simulink library "Camera_Frame_Definitions"  (R2025a)
settings: Solver=VariableStepAuto  StartTime=0.0  StopTime=10.0  RelTol=1e-3
values from neighbouring files (symbols this model uses):
  Camera = sm_car_define_camera(camera_param)    [sm_car_define_camera_sedan.m]
undefined symbols (not defined in the file or in its folder): X, Y, Z
libraries: sm_lib x40, $bdroot x30, nesl_utility x3
Description:
  | Component of Simscape Vehicle Templates Library
  | 
  | Copyright 2018-2026 The MathWorks, Inc.
settings Model: Creator=smiller  LastModifiedBy=smiller
settings SolverCC: AlgebraicLoopSolver=TrustRegion
settings DataIOCC: ReturnWorkspaceOutputs=off
settings OptimizationCC: LifeSpan=inf
settings DebuggingCC: UnconnectedInputMsg=warning  UnconnectedOutputMsg=warning  UnconnectedLineMsg=warning  SFExecutionAtInitializationDiag=none  ArithmeticOperatorsInVariantConditions=warning
settings ModelReferenceCC: EnableRefExpFcnMdlSchedulingChecks=on
settings SFSimCC: CustomCodeUndefinedFunction=UseInterfaceOnly
settings RTWCC: GPUComputeCapability=3.5
settings CodeAppCC: StateflowObjectComments=on

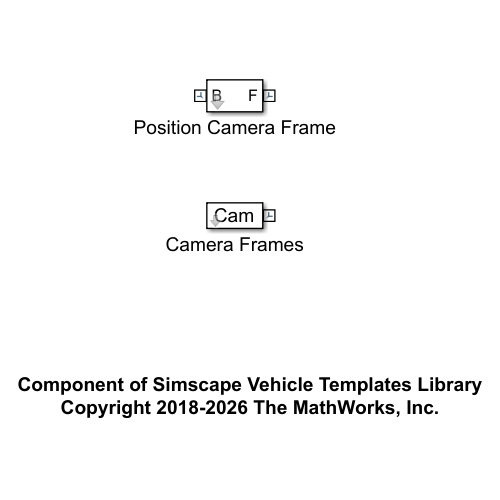
[thumbnail: Simulink's stored preview of the top-level diagram]
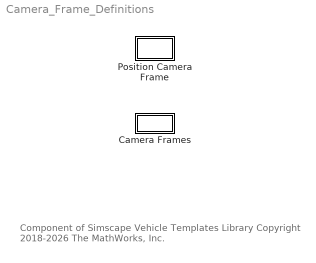
== system Camera_Frame_Definitions ==
  note: Component of Simscape Vehicle Templates Library
      | Copyright 2018-2026 The MathWorks, Inc.
  Camera Frames : Subsystem  mask(Camera Frame Definitions){Camera=Camera, popup_dolly_camera=Off}
      mask prompts: popup_dolly_camera "Dolly Camera"
      mask help: Defines set of camera frames surrounding vehicle. Frames are used to define visualization viewpoints for animation of simulation results.
      mask init:
      | if(verLessThan('matlab','9.5'))
      |   set_param([gcb '/Dolly Camera'],'OverrideUsingVariant',get_param(gcb,'popup_dolly_camera'));
      | else
      |   set_param([gcb '/Dolly Camera'],'LabelModeActiveChoice',get_param(gcb,'popup_dolly_camera'));
      | end
      mask TypeOptions popup_dolly_camera: Off | XYZ
      mask Display: disp('Cam')
  Position Camera Frame : Subsystem  mask(Define Camera Frame){CF=Camera.Rear}
      mask prompts: CF "Camera Frame Data (structure)"
      mask help: Sets frame position and orientation for camera frame. Data structure provides cartesian location and orientation. Orientation is intrinsic rotation of yaw-pitch-roll.

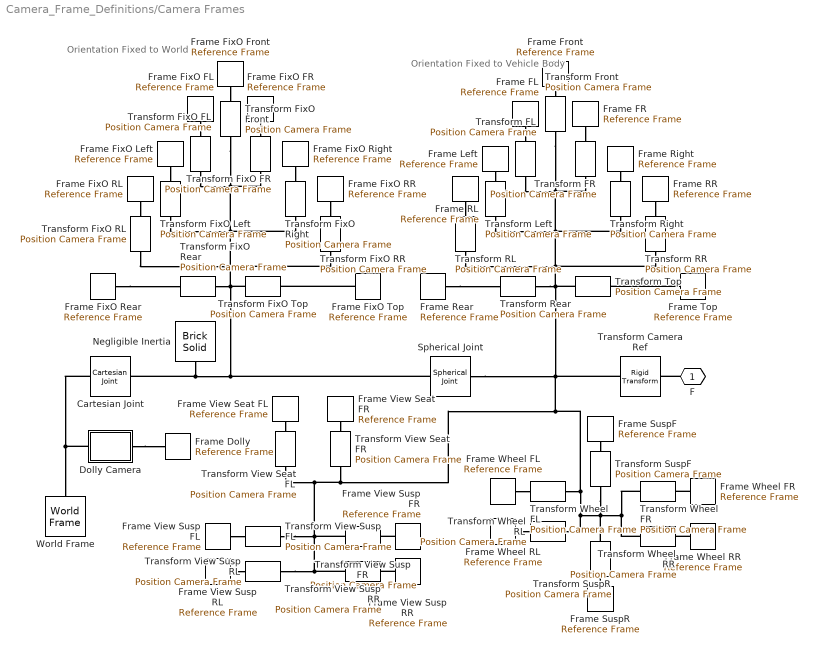
== system Camera_Frame_Definitions/Camera Frames ==
  note: Orientation Fixed to Vehicle Body
  note: Orientation Fixed to World
  Cartesian Joint : sm_lib/Joints/Cartesian Joint  JointMode=Normal  CompositeWrenchDir=FollowerOnBase  CompositeWrenchFrame=BaseFrame  SenseConstraintForce=off  SenseConstraintTorque=off  SenseTotalForce=off  SenseTotalTorque=off  PxPositionTargetSpecify=off  PxPositionTargetPriority=High  PxPositionTargetValue=0  PxPositionTargetValueUnits=m  PxVelocityTargetSpecify=off  PxVelocityTargetPriority=High  PxVelocityTargetValue=0  PxVelocityTargetValueUnits=m/s  PxEquilibriumPosition=0  PxEquilibriumPositionUnits=m  PxSpringStiffness=0  PxSpringStiffnessUnits=N/m  PxDampingCoefficient=0  PxDampingCoefficientUnits=N/(m/s)  PxLowerLimitSpecify=off  PxLowerLimitBound=-1  PxLowerLimitBoundUnits=m  PxLowerLimitStiffness=1e6  PxLowerLimitStiffnessUnits=N/m  PxLowerLimitDamping=1e3  PxLowerLimitDampingUnits=N/(m/s)  PxLowerLimitTransitionRegionWidth=1e-4  PxLowerLimitTransitionRegionWidthUnits=m  PxUpperLimitSpecify=off  PxUpperLimitBound=1  PxUpperLimitBoundUnits=m  PxUpperLimitStiffness=1e6  PxUpperLimitStiffnessUnits=N/m  PxUpperLimitDamping=1e3  PxUpperLimitDampingUnits=N/(m/s)  PxUpperLimitTransitionRegionWidth=1e-4  PxUpperLimitTransitionRegionWidthUnits=m  PxTorqueActuationMode=NoTorque  PxMotionActuationMode=ComputedMotion  PxSensePosition=off  PxSenseVelocity=off  PxSenseAcceleration=off  PxSenseTorqueForce=off  PxSenseLowerLimitTorqueForce=off  PxSenseUpperLimitTorqueForce=off  PyPositionTargetSpecify=off  PyPositionTargetPriority=High  PyPositionTargetValue=0  PyPositionTargetValueUnits=m  PyVelocityTargetSpecify=off  PyVelocityTargetPriority=High  PyVelocityTargetValue=0  PyVelocityTargetValueUnits=m/s  PyEquilibriumPosition=0  PyEquilibriumPositionUnits=m  PySpringStiffness=0  PySpringStiffnessUnits=N/m  PyDampingCoefficient=0  PyDampingCoefficientUnits=N/(m/s)  PyLowerLimitSpecify=off  PyLowerLimitBound=-1  PyLowerLimitBoundUnits=m  PyLowerLimitStiffness=1e6  PyLowerLimitStiffnessUnits=N/m  PyLowerLimitDamping=1e3  PyLowerLimitDampingUnits=N/(m/s)  PyLowerLimitTransitionRegionWidth=1e-4  PyLowerLimitTransitionRegionWidthUnits=m  PyUpperLimitSpecify=off  PyUpperLimitBound=1  PyUpperLimitBoundUnits=m  PyUpperLimitStiffness=1e6  PyUpperLimitStiffnessUnits=N/m  PyUpperLimitDamping=1e3  PyUpperLimitDampingUnits=N/(m/s)  PyUpperLimitTransitionRegionWidth=1e-4  PyUpperLimitTransitionRegionWidthUnits=m  PyTorqueActuationMode=NoTorque  PyMotionActuationMode=ComputedMotion  PySensePosition=off  PySenseVelocity=off  PySenseAcceleration=off  PySenseTorqueForce=off  PySenseLowerLimitTorqueForce=off  PySenseUpperLimitTorqueForce=off  PzPositionTargetSpecify=off  PzPositionTargetPriority=High  PzPositionTargetValue=0  PzPositionTargetValueUnits=m  PzVelocityTargetSpecify=off  PzVelocityTargetPriority=High  PzVelocityTargetValue=0  PzVelocityTargetValueUnits=m/s  PzEquilibriumPosition=0  PzEquilibriumPositionUnits=m  PzSpringStiffness=0  PzSpringStiffnessUnits=N/m  PzDampingCoefficient=0  PzDampingCoefficientUnits=N/(m/s)  PzLowerLimitSpecify=off  PzLowerLimitBound=-1  PzLowerLimitBoundUnits=m  PzLowerLimitStiffness=1e6  PzLowerLimitStiffnessUnits=N/m  PzLowerLimitDamping=1e3  PzLowerLimitDampingUnits=N/(m/s)  PzLowerLimitTransitionRegionWidth=1e-4  PzLowerLimitTransitionRegionWidthUnits=m  PzUpperLimitSpecify=off  PzUpperLimitBound=1  PzUpperLimitBoundUnits=m  PzUpperLimitStiffness=1e6  PzUpperLimitStiffnessUnits=N/m  PzUpperLimitDamping=1e3  PzUpperLimitDampingUnits=N/(m/s)  PzUpperLimitTransitionRegionWidth=1e-4  PzUpperLimitTransitionRegionWidthUnits=m  PzTorqueActuationMode=NoTorque  PzMotionActuationMode=ComputedMotion  PzSensePosition=off  PzSenseVelocity=off  PzSenseAcceleration=off  PzSenseTorqueForce=off  PzSenseLowerLimitTorqueForce=off  PzSenseUpperLimitTorqueForce=off
  Dolly Camera : Subsystem  Variant=on  VariantControlMode=label  VariantControl=Variant1  LabelModeActiveChoice=Off
      settings: AttributesFormatString=%<ActiveVariant>
      mask Display: disp(' ');
  Frame Dolly : sm_lib/Frames and Transforms/Reference Frame
  Frame FL : sm_lib/Frames and Transforms/Reference Frame
  Frame FR : sm_lib/Frames and Transforms/Reference Frame
  Frame FixO FL : sm_lib/Frames and Transforms/Reference Frame
  Frame FixO FR : sm_lib/Frames and Transforms/Reference Frame
  Frame FixO Front : sm_lib/Frames and Transforms/Reference Frame
  Frame FixO Left : sm_lib/Frames and Transforms/Reference Frame
  Frame FixO RL : sm_lib/Frames and Transforms/Reference Frame
  Frame FixO RR : sm_lib/Frames and Transforms/Reference Frame
  Frame FixO Rear : sm_lib/Frames and Transforms/Reference Frame
  Frame FixO Right : sm_lib/Frames and Transforms/Reference Frame
  Frame FixO Top : sm_lib/Frames and Transforms/Reference Frame
  Frame Front : sm_lib/Frames and Transforms/Reference Frame
  Frame Left : sm_lib/Frames and Transforms/Reference Frame
  Frame RL : sm_lib/Frames and Transforms/Reference Frame
  Frame RR : sm_lib/Frames and Transforms/Reference Frame
  Frame Rear : sm_lib/Frames and Transforms/Reference Frame
  Frame Right : sm_lib/Frames and Transforms/Reference Frame
  Frame SuspF : sm_lib/Frames and Transforms/Reference Frame
  Frame SuspR : sm_lib/Frames and Transforms/Reference Frame
  Frame Top : sm_lib/Frames and Transforms/Reference Frame
  Frame View Seat FL : sm_lib/Frames and Transforms/Reference Frame
  Frame View Seat FR : sm_lib/Frames and Transforms/Reference Frame
  Frame View Susp FL : sm_lib/Frames and Transforms/Reference Frame
  Frame View Susp FR : sm_lib/Frames and Transforms/Reference Frame
  Frame View Susp RL : sm_lib/Frames and Transforms/Reference Frame
  Frame View Susp RR : sm_lib/Frames and Transforms/Reference Frame
  Frame Wheel FL : sm_lib/Frames and Transforms/Reference Frame
  Frame Wheel FR : sm_lib/Frames and Transforms/Reference Frame
  Frame Wheel RL : sm_lib/Frames and Transforms/Reference Frame
  Frame Wheel RR : sm_lib/Frames and Transforms/Reference Frame
  Negligible Inertia : sm_lib/Body Elements/Brick Solid  BrickDimensions=[1 1 1]*1e-3  BrickDimensionsUnits=m  ExportEntireGeometry=off  InertiaType=PointMass  BasedOnType=Density  Density=1000  DensityUnits=kg/m^3  Mass=1e-6  MassUnits=kg  CenterOfMass=[0 0 0]  CenterOfMassUnits=m  MomentsOfInertia=[1 1 1]  MomentsOfInertiaUnits=kg*m^2  ProductsOfInertia=[1 1 1]  ProductsOfInertiaUnits=kg*m^2  GraphicType=FromGeometry  MarkerShape=Sphere  MarkerSize=10  GraphicVisPropType=SimpleVisualProperties  GraphicDiffuseColor=[0.5 0.5 0.5]  GraphicOpacity=1.0  GraphicSpecularColor=[0.5 0.5 0.5 1.0]  GraphicAmbientColor=[0.15 0.15 0.15 1.0]  GraphicEmissiveColor=[0.0 0.0 0.0 1.0]  GraphicShininess=75  DoExposeReferenceFrame=on  SerializedFrames=<Frames/>
  Spherical Joint : sm_lib/Joints/Spherical Joint  JointMode=Normal  CompositeWrenchDir=FollowerOnBase  CompositeWrenchFrame=BaseFrame  SenseConstraintForce=off  SenseConstraintTorque=off  SenseTotalForce=off  SenseTotalTorque=off  PositionTargetSpecify=off  PositionTargetPriority=High  PositionTargetRotationMethod=None  PositionTargetFollAlignAxisA=+X  PositionTargetBaseAlignAxisA=+Y  PositionTargetFollAlignAxisB=+Y  PositionTargetBaseAlignAxisB=+Z  PositionTargetRotationStandardAxis=+Z  PositionTargetRotationAngle=0.0  PositionTargetRotationAngleUnits=deg  PositionTargetRotationArbitraryAxis=[0 0 1]  PositionTargetRotationSequenceAxes=FollowerAxes  PositionTargetRotationSequence=XYX  PositionTargetRotationSequenceAngles=[0 0 0]  PositionTargetRotationSequenceAnglesUnits=deg  PositionTargetRotationMatrix=[1 0 0; 0 1 0; 0 0 1]  PositionTargetQuaternion=[1 0 0 0]  VelocityTargetSpecify=off  VelocityTargetPriority=High  VelocityTargetValue=[0 0 0]  VelocityTargetValueUnits=deg/s  VelocityTargetInFollowerFrame=on  EqPosRotationMethod=None  EqPosFollAlignAxisA=+X  EqPosBaseAlignAxisA=+Y  EqPosFollAlignAxisB=+Y  EqPosBaseAlignAxisB=+Z  EqPosRotationStandardAxis=+Z  EqPosRotationAngle=0.0  EqPosRotationAngleUnits=deg  EqPosRotationArbitraryAxis=[0 0 1]  EqPosRotationSequenceAxes=FollowerAxes  EqPosRotationSequence=XYX  EqPosRotationSequenceAngles=[0 0 0]  EqPosRotationSequenceAnglesUnits=deg  EqPosRotationMatrix=[1 0 0; 0 1 0; 0 0 1]  EqPosQuaternion=[1 0 0 0]  SpringStiffness=0  SpringStiffnessUnits=N*m/deg  DampingCoefficient=0  DampingCoefficientUnits=N*m/(deg/s)  LowerLimitSpecify=off  LowerLimitBound=15  LowerLimitBoundUnits=deg  LowerLimitStiffness=1e4  LowerLimitStiffnessUnits=N*m/deg  LowerLimitDamping=10  LowerLimitDampingUnits=N*m/(deg/s)  LowerLimitTransitionRegionWidth=0.1  LowerLimitTransitionRegionWidthUnits=deg  UpperLimitSpecify=off  UpperLimitBound=45  UpperLimitBoundUnits=deg  UpperLimitStiffness=1e4  UpperLimitStiffnessUnits=N*m/deg  UpperLimitDamping=10  UpperLimitDampingUnits=N*m/(deg/s)  UpperLimitTransitionRegionWidth=0.1  UpperLimitTransitionRegionWidthUnits=deg  TorqueActuationMode=NoTorque  ActuateTorqueX=off  ActuateTorqueY=off  ActuateTorqueZ=off  ActuateTorque=off  ActuationFrame=BaseFrame  SensePosition=off  SenseVelocityX=off  SenseVelocityY=off  SenseVelocityZ=off  SenseVelocity=off  SenseAccelerationX=off  SenseAccelerationY=off  SenseAccelerationZ=off  SenseAcceleration=off  SenseLowerLimitTorqueMag=off  SenseUpperLimitTorqueMag=off  SensingFrame=BaseFrame
  Transform Camera Ref : sm_lib/Frames and Transforms/Rigid Transform  RotationMethod=RotationSequence  FollAlignAxisA=+X  BaseAlignAxisA=+Y  FollAlignAxisB=+Y  BaseAlignAxisB=+Z  RotationStandardAxis=+Z  RotationAngle=0.0  RotationAngleUnits=deg  RotationArbitraryAxis=[0 0 1]  RotationSequenceAxes=FollowerAxes  RotationSequence=ZYX  RotationSequenceAngles=[Camera.Offset.a.Value(3) Camera.Offset.a.Value(2) Camera.Offset.a.Value(1)]  RotationSequenceAnglesUnits=deg  RotationMatrix=[1 0 0; 0 1 0; 0 0 1]  Quaternion=[1 0 0 0]  TranslationMethod=Cartesian  TranslationCartesianOffset=Camera.Offset.s.Value  TranslationCartesianOffsetUnits=m  TranslationStandardAxis=+Z  TranslationStandardOffset=0  TranslationStandardOffsetUnits=m  TranslationROffset=0  TranslationROffsetUnits=m  TranslationThetaOffset=0  TranslationThetaOffsetUnits=deg  TranslationZOffset=0  TranslationZOffsetUnits=m
  Transform FL : $bdroot/Position Camera Frame  CF=Camera.FL
  Transform FR : $bdroot/Position Camera Frame  CF=Camera.FR
  Transform FixO FL : $bdroot/Position Camera Frame  CF=Camera.FL
  Transform FixO FR : $bdroot/Position Camera Frame  CF=Camera.FR
  Transform FixO Front : $bdroot/Position Camera Frame  CF=Camera.Front
  Transform FixO Left : $bdroot/Position Camera Frame  CF=Camera.Left
  Transform FixO RL : $bdroot/Position Camera Frame  CF=Camera.RL
  Transform FixO RR : $bdroot/Position Camera Frame  CF=Camera.RR
  Transform FixO Rear : $bdroot/Position Camera Frame  CF=Camera.Rear
  Transform FixO Right : $bdroot/Position Camera Frame  CF=Camera.Right
  Transform FixO Top : $bdroot/Position Camera Frame  CF=Camera.Top
  Transform Front : $bdroot/Position Camera Frame  CF=Camera.Front
  Transform Left : $bdroot/Position Camera Frame  CF=Camera.Left
  Transform RL : $bdroot/Position Camera Frame  CF=Camera.RL
  Transform RR : $bdroot/Position Camera Frame  CF=Camera.RR
  Transform Rear : $bdroot/Position Camera Frame  CF=Camera.Rear
  Transform Right : $bdroot/Position Camera Frame  CF=Camera.Right
  Transform SuspF : $bdroot/Position Camera Frame  CF=Camera.SuspF
  Transform SuspR : $bdroot/Position Camera Frame  CF=Camera.SuspR
  Transform Top : $bdroot/Position Camera Frame  CF=Camera.Top
  Transform View Seat FL : $bdroot/Position Camera Frame  CF=Camera.View_SeatFL
  Transform View Seat FR : $bdroot/Position Camera Frame  CF=Camera.View_SeatFR
  Transform View Susp FL : $bdroot/Position Camera Frame  CF=Camera.View_SuspFL
  Transform View Susp FR : $bdroot/Position Camera Frame  CF=Camera.View_SuspFR
  Transform View Susp RL : $bdroot/Position Camera Frame  CF=Camera.View_SuspRL
  Transform View Susp RR : $bdroot/Position Camera Frame  CF=Camera.View_SuspRR
  Transform Wheel FL : $bdroot/Position Camera Frame  CF=Camera.Wheel_FL
  Transform Wheel FR : $bdroot/Position Camera Frame  CF=Camera.Wheel_FR
  Transform Wheel RL : $bdroot/Position Camera Frame  CF=Camera.Wheel_RL
  Transform Wheel RR : $bdroot/Position Camera Frame  CF=Camera.Wheel_RR
  World Frame : sm_lib/Frames and Transforms/World Frame
  F : PMIOPort  Side=Right
  connections:
  F/RConn1 -- Transform Camera Ref/LConn1
  Transform View Susp FR/LConn1 -- Transform View Susp RL/LConn1 -- Transform View Susp RR/LConn1 -- Transform View Seat FR/LConn1 -- Transform Wheel RR/LConn1 -- Transform Wheel FR/LConn1 -- Transform SuspR/LConn1 -- Transform SuspF/LConn1 -- Transform Wheel RL/LConn1 -- Transform Wheel FL/LConn1 -- Spherical Joint/RConn1 -- Transform Camera Ref/RConn1 -- Transform Top/LConn1 -- Transform RL/LConn1 -- Transform RR/LConn1 -- Transform Left/LConn1 -- Transform Right/LConn1 -- Transform FR/LConn1 -- Transform Front/LConn1 -- Transform FL/LConn1 -- Transform Rear/LConn1 -- Transform View Seat FL/LConn1 -- Transform View Susp FL/LConn1
  Dolly Camera/LConn1 -- Cartesian Joint/LConn1 -- World Frame/RConn1
  Negligible Inertia/RConn1 -- Cartesian Joint/RConn1 -- Spherical Joint/LConn1 -- Transform FixO Rear/LConn1 -- Transform FixO Top/LConn1 -- Transform FixO FL/LConn1 -- Transform FixO Front/LConn1 -- Transform FixO FR/LConn1 -- Transform FixO Right/LConn1 -- Transform FixO Left/LConn1 -- Transform FixO RR/LConn1 -- Transform FixO RL/LConn1
  Frame FixO FR/RConn1 -- Transform FixO FR/RConn1
  Frame FixO Right/RConn1 -- Transform FixO Right/RConn1
  Frame FixO RR/RConn1 -- Transform FixO RR/RConn1
  Frame FixO RL/RConn1 -- Transform FixO RL/RConn1
  Frame FixO Left/RConn1 -- Transform FixO Left/RConn1
  Frame FixO FL/RConn1 -- Transform FixO FL/RConn1
  Frame FixO Top/RConn1 -- Transform FixO Top/RConn1
  Frame FixO Front/RConn1 -- Transform FixO Front/RConn1
  Frame FixO Rear/RConn1 -- Transform FixO Rear/RConn1
  Frame Rear/RConn1 -- Transform Rear/RConn1
  Frame Top/RConn1 -- Transform Top/RConn1
  Frame Left/RConn1 -- Transform Left/RConn1
  Frame FL/RConn1 -- Transform FL/RConn1
  Frame RL/RConn1 -- Transform RL/RConn1
  Frame Right/RConn1 -- Transform Right/RConn1
  Frame FR/RConn1 -- Transform FR/RConn1
  Frame RR/RConn1 -- Transform RR/RConn1
  Frame Front/RConn1 -- Transform Front/RConn1
  Frame SuspF/RConn1 -- Transform SuspF/RConn1
  Frame SuspR/RConn1 -- Transform SuspR/RConn1
  Frame Wheel FR/RConn1 -- Transform Wheel FR/RConn1
  Frame Wheel RR/RConn1 -- Transform Wheel RR/RConn1
  Frame Wheel FL/RConn1 -- Transform Wheel FL/RConn1
  Frame Wheel RL/RConn1 -- Transform Wheel RL/RConn1
  Frame View Seat FL/RConn1 -- Transform View Seat FL/RConn1
  Frame View Seat FR/RConn1 -- Transform View Seat FR/RConn1
  Frame View Susp FL/RConn1 -- Transform View Susp FL/RConn1
  Frame View Susp FR/RConn1 -- Transform View Susp FR/RConn1
  Frame View Susp RR/RConn1 -- Transform View Susp RR/RConn1
  Frame View Susp RL/RConn1 -- Transform View Susp RL/RConn1
  Dolly Camera/RConn1 -- Frame Dolly/RConn1

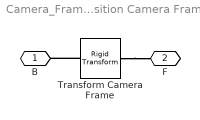
== system Camera_Frame_Definitions/Position Camera Frame ==
  Transform Camera Frame : sm_lib/Frames and Transforms/Rigid Transform  RotationMethod=RotationSequence  FollAlignAxisA=+X  BaseAlignAxisA=+Y  FollAlignAxisB=+Y  BaseAlignAxisB=+Z  RotationStandardAxis=+Z  RotationAngle=0.0  RotationAngleUnits=deg  RotationArbitraryAxis=[0 0 1]  RotationSequenceAxes=FollowerAxes  RotationSequence=ZYX  RotationSequenceAngles=CF.a.Value(3:-1:1)  RotationSequenceAnglesUnits=deg  RotationMatrix=[1 0 0; 0 1 0; 0 0 1]  Quaternion=[1 0 0 0]  TranslationMethod=Cartesian  TranslationCartesianOffset=CF.s.Value  TranslationCartesianOffsetUnits=m  TranslationStandardAxis=+Z  TranslationStandardOffset=0  TranslationStandardOffsetUnits=m  TranslationROffset=0  TranslationROffsetUnits=m  TranslationThetaOffset=0  TranslationThetaOffsetUnits=deg  TranslationZOffset=0  TranslationZOffsetUnits=m
  B : PMIOPort  Side=Left
  F : PMIOPort  Port=2  Side=Right
  connections:
  Transform Camera Frame/LConn1 -- B/RConn1
  Transform Camera Frame/RConn1 -- F/RConn1

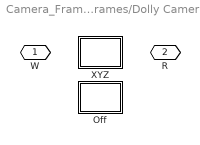
== system Camera_Frame_Definitions/Camera Frames/Dolly Camera ==
  Off : Subsystem  VariantControl=Off  mask{tvec=Camera.Dolly_Cam.tvec.Value, xvec=Camera.Dolly_Cam.xvec.Value, yvec=Camera.Dolly_Cam.yvec.Value, zvec=Camera.Dolly_Cam.zvec.Value, s=Camera.Dolly_Cam.s.Value, a=Camera.Dolly_Cam.a.Value}
      mask prompts: tvec "Time Vector (s)"; xvec "X Vector (m)"; yvec "Y Vector (m)"; zvec "Z Vector (m)"; s "Camera Offset [xyz] (m)"; a "Camera Orientation [Roll-Pitch-Yaw] (deg)"
  XYZ : Subsystem  VariantControl=XYZ  mask{tvec=Camera.Dolly_Cam.tvec.Value, xvec=Camera.Dolly_Cam.xvec.Value, yvec=Camera.Dolly_Cam.yvec.Value, zvec=Camera.Dolly_Cam.zvec.Value, s=Camera.Dolly_Cam.s.Value, a=Camera.Dolly_Cam.a.Value}
      mask prompts: tvec "Time Vector (s)"; xvec "X Vector (m)"; yvec "Y Vector (m)"; zvec "Z Vector (m)"; s "Camera Offset [xyz] (m)"; a "Camera Orientation [Roll-Pitch-Yaw] (deg)"
  " W" : PMIOPort  Side=Left
  " R" : PMIOPort  Port=2  Side=Right

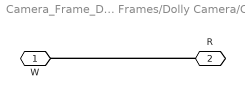
== system Camera_Frame_Definitions/Camera Frames/Dolly Camera/Off ==
  W : PMIOPort  Side=Left
  R : PMIOPort  Port=2  Side=Right
  connections:
  R/RConn1 -- W/RConn1

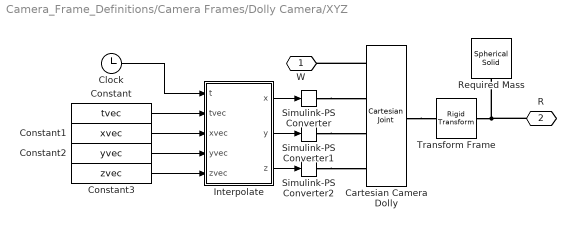
== system Camera_Frame_Definitions/Camera Frames/Dolly Camera/XYZ ==
  Cartesian Camera Dolly : sm_lib/Joints/Cartesian Joint  JointMode=Normal  CompositeWrenchDir=FollowerOnBase  CompositeWrenchFrame=BaseFrame  SenseConstraintForce=off  SenseConstraintTorque=off  SenseTotalForce=off  SenseTotalTorque=off  PxPositionTargetSpecify=on  PxPositionTargetPriority=High  PxPositionTargetValue=xvec(1)  PxPositionTargetValueUnits=m  PxVelocityTargetSpecify=off  PxVelocityTargetPriority=High  PxVelocityTargetValue=0  PxVelocityTargetValueUnits=m/s  PxEquilibriumPosition=0  PxEquilibriumPositionUnits=m  PxSpringStiffness=0  PxSpringStiffnessUnits=N/m  PxDampingCoefficient=0  PxDampingCoefficientUnits=N/(m/s)  PxLowerLimitSpecify=off  PxLowerLimitBound=-1  PxLowerLimitBoundUnits=m  PxLowerLimitStiffness=1e6  PxLowerLimitStiffnessUnits=N/m  PxLowerLimitDamping=1e3  PxLowerLimitDampingUnits=N/(m/s)  PxLowerLimitTransitionRegionWidth=1e-4  PxLowerLimitTransitionRegionWidthUnits=m  PxUpperLimitSpecify=off  PxUpperLimitBound=1  PxUpperLimitBoundUnits=m  PxUpperLimitStiffness=1e6  PxUpperLimitStiffnessUnits=N/m  PxUpperLimitDamping=1e3  PxUpperLimitDampingUnits=N/(m/s)  PxUpperLimitTransitionRegionWidth=1e-4  PxUpperLimitTransitionRegionWidthUnits=m  PxTorqueActuationMode=ComputedTorque  PxMotionActuationMode=InputMotion  PxSensePosition=off  PxSenseVelocity=off  PxSenseAcceleration=off  PxSenseTorqueForce=off  PxSenseLowerLimitTorqueForce=off  PxSenseUpperLimitTorqueForce=off  PyPositionTargetSpecify=on  PyPositionTargetPriority=High  PyPositionTargetValue=yvec(1)  PyPositionTargetValueUnits=m  PyVelocityTargetSpecify=off  PyVelocityTargetPriority=High  PyVelocityTargetValue=0  PyVelocityTargetValueUnits=m/s  PyEquilibriumPosition=0  PyEquilibriumPositionUnits=m  PySpringStiffness=0  PySpringStiffnessUnits=N/m  PyDampingCoefficient=0  PyDampingCoefficientUnits=N/(m/s)  PyLowerLimitSpecify=off  PyLowerLimitBound=-1  PyLowerLimitBoundUnits=m  PyLowerLimitStiffness=1e6  PyLowerLimitStiffnessUnits=N/m  PyLowerLimitDamping=1e3  PyLowerLimitDampingUnits=N/(m/s)  PyLowerLimitTransitionRegionWidth=1e-4  PyLowerLimitTransitionRegionWidthUnits=m  PyUpperLimitSpecify=off  PyUpperLimitBound=1  PyUpperLimitBoundUnits=m  PyUpperLimitStiffness=1e6  PyUpperLimitStiffnessUnits=N/m  PyUpperLimitDamping=1e3  PyUpperLimitDampingUnits=N/(m/s)  PyUpperLimitTransitionRegionWidth=1e-4  PyUpperLimitTransitionRegionWidthUnits=m  PyTorqueActuationMode=ComputedTorque  PyMotionActuationMode=InputMotion  PySensePosition=off  PySenseVelocity=off  PySenseAcceleration=off  PySenseTorqueForce=off  PySenseLowerLimitTorqueForce=off  PySenseUpperLimitTorqueForce=off  PzPositionTargetSpecify=on  PzPositionTargetPriority=High  PzPositionTargetValue=zvec(1)  PzPositionTargetValueUnits=m  PzVelocityTargetSpecify=off  PzVelocityTargetPriority=High  PzVelocityTargetValue=0  PzVelocityTargetValueUnits=m/s  PzEquilibriumPosition=0  PzEquilibriumPositionUnits=m  PzSpringStiffness=0  PzSpringStiffnessUnits=N/m  PzDampingCoefficient=0  PzDampingCoefficientUnits=N/(m/s)  PzLowerLimitSpecify=off  PzLowerLimitBound=-1  PzLowerLimitBoundUnits=m  PzLowerLimitStiffness=1e6  PzLowerLimitStiffnessUnits=N/m  PzLowerLimitDamping=1e3  PzLowerLimitDampingUnits=N/(m/s)  PzLowerLimitTransitionRegionWidth=1e-4  PzLowerLimitTransitionRegionWidthUnits=m  PzUpperLimitSpecify=off  PzUpperLimitBound=1  PzUpperLimitBoundUnits=m  PzUpperLimitStiffness=1e6  PzUpperLimitStiffnessUnits=N/m  PzUpperLimitDamping=1e3  PzUpperLimitDampingUnits=N/(m/s)  PzUpperLimitTransitionRegionWidth=1e-4  PzUpperLimitTransitionRegionWidthUnits=m  PzTorqueActuationMode=ComputedTorque  PzMotionActuationMode=InputMotion  PzSensePosition=off  PzSenseVelocity=off  PzSenseAcceleration=off  PzSenseTorqueForce=off  PzSenseLowerLimitTorqueForce=off  PzSenseUpperLimitTorqueForce=off
  Clock : Clock
  Constant : Constant  Value=tvec
  Constant1 : Constant  Value=xvec
  Constant2 : Constant  Value=yvec
  Constant3 : Constant  Value=zvec
  Interpolate : MATLAB Function  TreatAsAtomicUnit=on
  Required Mass : sm_lib/Body Elements/Spherical Solid  SphereRadius=0.05  SphereRadiusUnits=m  ExportEntireGeometry=off  InertiaType=CalculateFromGeometry  BasedOnType=Density  Density=1000  DensityUnits=kg/m^3  Mass=1  MassUnits=kg  CenterOfMass=[0 0 0]  CenterOfMassUnits=m  MomentsOfInertia=[1 1 1]  MomentsOfInertiaUnits=kg*m^2  ProductsOfInertia=[0 0 0]  ProductsOfInertiaUnits=kg*m^2  GraphicType=FromGeometry  MarkerShape=Sphere  MarkerSize=10  GraphicVisPropType=SimpleVisualProperties  GraphicDiffuseColor=[0.2 1.0 0.0]  GraphicOpacity=0  GraphicSpecularColor=[0.5 0.5 0.5 1.0]  GraphicAmbientColor=[0.15 0.15 0.15 1.0]  GraphicEmissiveColor=[0.0 0.0 0.0 1.0]  GraphicShininess=75  DoExposeReferenceFrame=on  SerializedFrames=<Frames/>
  Simulink-PS Converter : nesl_utility/Simulink-PS Converter  PhysicalDomain=network_engine_domain  SubClassName=ps_input  LeftPortType=input  RightPortType=output  PseudoPeriodic=off  Frequencies=[]  NoiseDistribution=none  NoiseParameters=[]  Unit=1  AffineConversion=off  FilteringAndDerivatives=filter  SimscapeFilterOrder=2  InputFilterTimeConstant=0.1  UdotUserProvided=1
  Simulink-PS Converter1 : nesl_utility/Simulink-PS Converter  PhysicalDomain=network_engine_domain  SubClassName=ps_input  LeftPortType=input  RightPortType=output  PseudoPeriodic=off  Frequencies=[]  NoiseDistribution=none  NoiseParameters=[]  Unit=1  AffineConversion=off  FilteringAndDerivatives=filter  SimscapeFilterOrder=2  InputFilterTimeConstant=0.1  UdotUserProvided=1
  Simulink-PS Converter2 : nesl_utility/Simulink-PS Converter  PhysicalDomain=network_engine_domain  SubClassName=ps_input  LeftPortType=input  RightPortType=output  PseudoPeriodic=off  Frequencies=[]  NoiseDistribution=none  NoiseParameters=[]  Unit=1  AffineConversion=off  FilteringAndDerivatives=filter  SimscapeFilterOrder=2  InputFilterTimeConstant=0.1  UdotUserProvided=1
  Transform Frame : sm_lib/Frames and Transforms/Rigid Transform  RotationMethod=RotationSequence  FollAlignAxisA=+X  BaseAlignAxisA=+Y  FollAlignAxisB=+Y  BaseAlignAxisB=+Z  RotationStandardAxis=+Z  RotationAngle=0.0  RotationAngleUnits=deg  RotationArbitraryAxis=[0 0 1]  RotationSequenceAxes=FollowerAxes  RotationSequence=ZYX  RotationSequenceAngles=a([3 2 1])  RotationSequenceAnglesUnits=deg  RotationMatrix=[1 0 0; 0 1 0; 0 0 1]  Quaternion=[1 0 0 0]  TranslationMethod=Cartesian  TranslationCartesianOffset=s  TranslationCartesianOffsetUnits=m  TranslationStandardAxis=+Z  TranslationStandardOffset=0  TranslationStandardOffsetUnits=m  TranslationROffset=0  TranslationROffsetUnits=m  TranslationThetaOffset=0  TranslationThetaOffsetUnits=deg  TranslationZOffset=0  TranslationZOffsetUnits=m
  W : PMIOPort  Side=Left
  R : PMIOPort  Port=2  Side=Right
  wires:
  Clock/1 -> Interpolate/1(t)
  Constant/1 -> Interpolate/2(tvec)
  Constant1/1 -> Interpolate/3(xvec)
  Interpolate/1(x) -> Simulink-PS Converter/1
  Interpolate/2(y) -> Simulink-PS Converter1/1
  Interpolate/3(z) -> Simulink-PS Converter2/1
  Constant2/1 -> Interpolate/4(yvec)
  Constant3/1 -> Interpolate/5(zvec)
  connections:
  Cartesian Camera Dolly/LConn1 -- W/RConn1
  Simulink-PS Converter/RConn1 -- Cartesian Camera Dolly/LConn2
  Transform Frame/RConn1 -- Required Mass/RConn1 -- R/RConn1
  Cartesian Camera Dolly/RConn1 -- Transform Frame/LConn1
  Simulink-PS Converter1/RConn1 -- Cartesian Camera Dolly/LConn3
  Simulink-PS Converter2/RConn1 -- Cartesian Camera Dolly/LConn4

== matlab function Camera_Frame_Definitions/Camera Frames/Dolly Camera/XYZ/Interpolate ==
  data: t input; x output; tvec input; xvec input; yvec input; zvec input; y output; z output
function [x,y,z] = fcn(t,tvec,xvec,yvec,zvec)

x = interp1(tvec,xvec,t,'pchip');
y = interp1(tvec,yvec,t,'pchip');
z = interp1(tvec,zvec,t,'pchip');
